simulink model "torpedo"  (R2024b)
settings: Solver=VariableStepAuto  StartTime=0.0  StopTime=10.0  RelTol=1e-3
libraries: dspnetwork x2, shared6dof x1
settings Model: Creator=gokde  LastModifiedBy=gokde

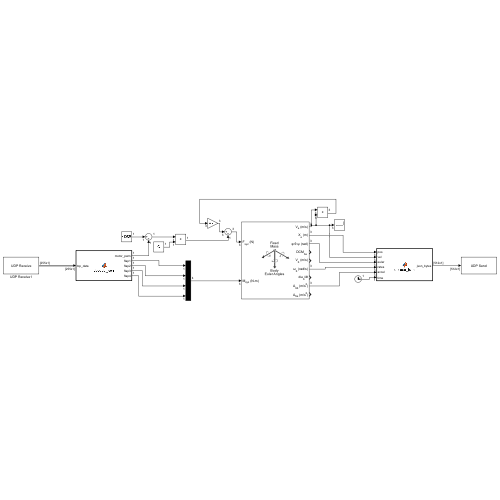
[thumbnail: Simulink's stored preview of the top-level diagram]
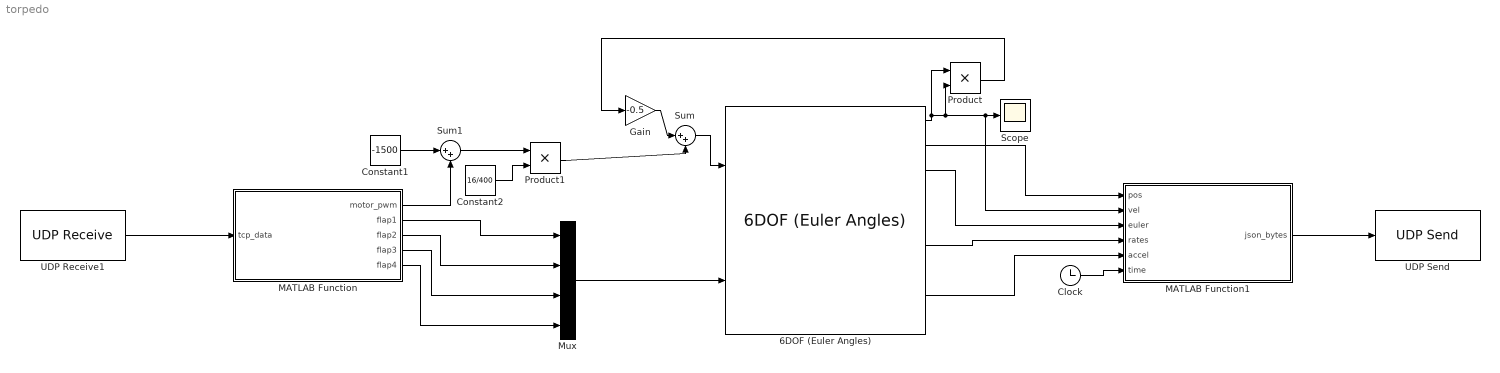
== system torpedo ==
  6DOF (Euler Angles) : shared6dof/6DOF (Euler Angles)  units=Metric (MKS)  mtype=Fixed  rep=Euler Angles  xme_0=[0 0 -10]  Vm_0=[0 0 0]  eul_0=[0 0 0]  pm_0=[0 0 0]  mass_0=5.0  mass_e=0.5  mass_f=2.0  inertia=[0.1 0 0; 0 0.5 0; 0 0 0.5]  inertia_e=eye(3)  inertia_f=2*eye(3)  k_quat=1.0  vre_flag=on  abi_flag=on  aMode=0  xme_statename=''  Vm_statename=''  eul_statename=''  quat_statename=''  pm_statename=''  mass_statename=''
  Clock : Clock
  Constant1 : Constant  Value=-1500
  Constant2 : Constant  Value=16/400
  Gain : Gain  Gain=-0.5
  MATLAB Function : MATLAB Function  TreatAsAtomicUnit=on
  MATLAB Function1 : MATLAB Function  TreatAsAtomicUnit=on
  Mux : Mux
  Product : Product
  Product1 : Product
  Scope : Scope
  Sum : Sum  Inputs=|++
  Sum1 : Sum  Inputs=|++
  UDP Receive1 : dspnetwork/UDP Receive  localURL='0.0.0.0'  localPort=9003  remoteURL='0.0.0.0'  remotePort=-1  recvBufferSize=8192  dims=255  signalDatatype=uint8  isComplex=off  isVarSize=on  showBlockingTime=off  blockingTime=0  sampletime=1  blockPlatform=[]
      settings: LibrarySourceBlock=dspsrcs4/UDP Receive
  UDP Send : dspnetwork/UDP Send  remoteURL='127.0.0.1'  remotePort=9002  localURL='0.0.0.0'  localPortSource=Automatically determine  localPort=-1  sendBufferSize=8192  sampletime=-1  blockPlatform=[]  separateLengthPort=0
      settings: LibrarySourceBlock=dspsnks4/UDP Send
  wires:
  6DOF (Euler Angles)/1 -> Product/1, Product/2, MATLAB Function1/2(vel), Scope/1
  Product/1 -> Gain/1
  Gain/1 -> Sum/1
  Sum/1 -> 6DOF (Euler Angles)/1
  MATLAB Function/1(motor_pwm) -> Sum1/2
  Constant1/1 -> Sum1/1
  Sum1/1 -> Product1/1
  Constant2/1 -> Product1/2
  Product1/1 -> Sum/2
  6DOF (Euler Angles)/2 -> MATLAB Function1/1(pos)
  6DOF (Euler Angles)/3 -> MATLAB Function1/3(euler)
  6DOF (Euler Angles)/6 -> MATLAB Function1/4(rates)
  6DOF (Euler Angles)/8 -> MATLAB Function1/5(accel)
  Clock/1 -> MATLAB Function1/6(time)
  UDP Receive1/1 -> MATLAB Function/1(tcp_data)
  MATLAB Function1/1(json_bytes) -> UDP Send/1
  MATLAB Function/2(flap1) -> Mux/1
  MATLAB Function/3(flap2) -> Mux/2
  MATLAB Function/4(flap3) -> Mux/3
  MATLAB Function/5(flap4) -> Mux/4
  Mux/1 -> 6DOF (Euler Angles)/2

== matlab function torpedo/MATLAB Function1 ==
  data: pos input; json_bytes output; vel input; euler input; rates input; accel input; time input
function json_bytes = encode_json(pos, vel, euler, rates, accel, time)
    % Bu fonksiyonun dışarıdan (MATLAB motorundan) çağrılacağını belirtiyoruz
    coder.extrinsic('jsonencode');

    % 1. Veri Paketini Oluştur
    packet = struct;
    packet.timestamp = time;
    
    % ArduPlane SITL formatı (Değerler double olmalı)
    packet.imu.gyro = rates; 
    packet.imu.accel_body = accel;
    
    % Konum (Basit düz dünya kabulü - İstanbul)
    lat_start = 41.0082;
    lon_start = 28.9784;
    
    % Derece dönüşümleri
    packet.position.lat = lat_start + (double(pos(1)) / 111111);
    packet.position.lon = lon_start + (double(pos(2)) / (111111 * cosd(lat_start)));
    packet.position.alt = -double(pos(3)); 
    
    packet.velocity.vx = double(vel(1));
    packet.velocity.vy = double(vel(2));
    packet.velocity.vz = double(vel(3));
    
    packet.attitude.roll = double(euler(1));
    packet.attitude.pitch = double(euler(2));
    packet.attitude.yaw = double(euler(3));

    % 2. JSON'a Çevir (Extrinsic Çağrı)
    % Simulink derleyicisi sonucun ne olacağını bilemez, bu yüzden
    % önce boş bir değişken tanımlamalıyız.
    str_temp = ''; 
    str_temp = jsonencode(packet);
    
    % 3. Boyutu Sabitle (ÇOK ÖNEMLİ)
    % TCP Bloğu sabit boyut ister (Örn: 512 byte).
    % JSON stringi kısa olsa bile sonunu sıfırla doldurmalıyız.
    
    json_bytes = zeros(512, 1, 'uint8'); % 512 byte'lık boş tampon
    
    % Stringi uint8 dizisine çevir
    raw_bytes = uint8(char(str_temp));
    
    % Veriyi tampona sığdır (Taşmayı önle)
    len = min(length(raw_bytes), 512);
    json_bytes(1:len) = raw_bytes(1:len);
end

== matlab function torpedo/MATLAB Function ==
  data: tcp_data input; motor_pwm output; flap1 output; flap2 output; flap3 output; flap4 output
function [motor_pwm, flap1, flap2, flap3, flap4] = decode_json(tcp_data)
    % str2num fonksiyonunu MATLAB motorunda çalıştıracağız
    coder.extrinsic('str2num');

    % 1. Varsayılan Değerler (Sinyal kesilirse saçmalamasın)
    motor_pwm = 1500;
    flap1 = 1500;
    flap2 = 1500;
    flap3 = 1500;
    flap4 = 1500;

    % 2. Veriyi Karaktere Çevir
    str = char(tcp_data');
    
    % 3. "servos" dizisini String işlemleriyle bul
    % ArduPlane verisi şöyledir: ... "servos":[1100, 1500, 1500, ...] ...
    
    key = '"servos":[';
    idx_start = strfind(str, key);
    
    if ~isempty(idx_start)
        % Köşeli parantezden sonrasını al
        % key'in uzunluğu 10 karakterdir, o yüzden +10 ekliyoruz
        data_start = idx_start(1) + 10;
        
        % Stringin geri kalanına bak
        remaining_str = str(data_start:end);
        
        % Kapanış parantezini ']' bul
        idx_end = strfind(remaining_str, ']');
        
        if ~isempty(idx_end)
            % Sadece sayıların olduğu kısmı kesip al (Örn: "1100, 1500, 1500")
            numbers_str = remaining_str(1:idx_end(1)-1);
            
            % 4. Stringi Sayı Dizisine Çevir
            % str2num, jsondecode gibi struct değil, "Matris" döndürür.
            % Simulink matrisleri extrinsic olsa bile anlayabilir.
            vals = str2num(numbers_str);
            
            % 5. Değerleri Ata
            if length(vals) >= 5
                motor_pwm = double(vals(1));
                flap1     = double(vals(2));
                flap2     = double(vals(3));
                flap3     = double(vals(4));
                flap4     = double(vals(5));
            end
        end
    end
end
